simulink model "sys1"  (R2023b)
settings: Solver=VariableStepAuto  StartTime=0.0  StopTime=30e-3  RelTol=1e-3
InitFcn:
  | fs = 100e6;
  | ts = 1 / fs;
values from neighbouring files (symbols this model uses):
  c = 3e8    (= 300000000)    [init_param.m]
  H_az1 = zeros(numSamples,numPulses)    [init_param.m]
  H_az2 = zeros(numSamples,numPulses)    [init_param.m]
  H_ref = fft(conj(fliplr(txChirp)), numSamples)    [init_param.m]
  rawData = rawData + 0.01 * (randn(size(rawData)) + 1j * randn(size(rawData)))    [init_param.m]
  x1 = zeros(size(rawData))    [main.m]
  x2 = zeros(size(x1))    [main.m]
  x3 = zeros(size(x2))    [main.m]
  x4 = zeros(size(x3))    [main.m]
  x5 = zeros(size(x4))    [main.m]
  x6 = zeros(size(x5))    [main.m]
  xx4 = zeros(size(xx3))    [main.m]
  xx5 = zeros(size(xx4))    [main.m]
  xx6 = zeros(size(xx5))    [main.m]
undefined symbols (not defined in the file or in its folder): ffva1156, w2, w3, w4, w5, w6, w7, w8, w9, ww2, ww3, ww4, ww5, ww6, ww7, ww8, ww9, xcku095
libraries: hdlBasic x917, hdlDSPIP x18, dspsrcs4 x12, vmcUtilities x1
(part 2 of 9)

== system sys1/SAR/stream/stream_ifft ==
  en : Inport
  re : Inport  Port=2
  im : Inport  Port=3
  Scale : hdlBasic/Scale  scale_factor=15  XmcBlockStatus=1  maskContainerNames=group1  block_type=scale  block_config=sysgen:Scale_config
  Scale1 : hdlBasic/Scale  scale_factor=15  XmcBlockStatus=1  maskContainerNames=group1  block_type=scale  block_config=sysgen:Scale_config
  Scale2 : hdlBasic/Scale  scale_factor=-15  XmcBlockStatus=1  maskContainerNames=group1  block_type=scale  block_config=sysgen:Scale_config
  Scale3 : hdlBasic/Scale  scale_factor=-15  XmcBlockStatus=1  maskContainerNames=group1  block_type=scale  block_config=sysgen:Scale_config
  stage1 : Subsystem
  stage2 : Subsystem
  stage3 : Subsystem
  stage4 : Subsystem
  stage5 : Subsystem
  stage6 : Subsystem
  stage7 : Subsystem
  stage8 : Subsystem
  stage9 : Subsystem
  valid : Outport
  out_re : Outport  Port=2
  out_im : Outport  Port=3
  wires:
  stage7/3(out_im) -> stage8/3(im)
  stage5/3(out_im) -> stage6/3(im)
  stage8/3(out_im) -> stage9/3(im)
  en/1 -> stage1/1(en)
  stage2/3(out_im) -> stage3/3(im)
  stage1/3(out_im) -> stage2/3(im)
  stage6/3(out_im) -> stage7/3(im)
  stage4/3(out_im) -> stage5/3(im)
  im/1 -> Scale1/1
  stage3/3(out_im) -> stage4/3(im)
  re/1 -> Scale/1
  stage9/3(out_im) -> Scale3/1
  stage1/1(valid) -> stage2/1(en)
  stage1/2(out_re) -> stage2/2(re)
  stage2/2(out_re) -> stage3/2(re)
  stage2/1(valid) -> stage3/1(en)
  stage3/1(valid) -> stage4/1(en)
  stage3/2(out_re) -> stage4/2(re)
  stage4/2(out_re) -> stage5/2(re)
  stage4/1(valid) -> stage5/1(en)
  stage5/1(valid) -> stage6/1(en)
  stage5/2(out_re) -> stage6/2(re)
  stage6/2(out_re) -> stage7/2(re)
  stage6/1(valid) -> stage7/1(en)
  stage7/1(valid) -> stage8/1(en)
  stage7/2(out_re) -> stage8/2(re)
  stage8/2(out_re) -> stage9/2(re)
  stage8/1(valid) -> stage9/1(en)
  stage9/1(valid) -> valid/1
  stage9/2(out_re) -> Scale2/1
  Scale/1 -> stage1/2(re)
  Scale1/1 -> stage1/3(im)
  Scale2/1 -> out_re/1
  Scale3/1 -> out_im/1

== system sys1/SAR/stream/stream_fft/stage1 ==
  en : Inport
  re : Inport  Port=2
  im : Inport  Port=3
  BF : Subsystem
      settings: PortSchema="{\"entries\":[{\"content\":{\"sides\":[{\"content\":{\"connectorIds\":[\"In1\",\"In2\",\"Out3\",\"Out4\"]},\"type\":\"ConnectorPlacement.EquallySpacedRectSide\",\"uuid\":\"dc9f2664-179f-4a56-867a-12fe61ba91e8\"},{\"content\":{\"connectorIds\":[\"Out1\",\"Out2\",\"In3\",\"In4\"],\"side\":\"RIGHT\"},\"type\":\"ConnectorPlacement.EquallySpacedRectSide\",\"uuid\":\"0b440064-4d1a-4bb1-bd44-91090294f336\"},{\"content\":{\"side\":\"TOP\"},\"type\":\"ConnectorPlacement.EquallySpacedRectSide\",\"uuid\":\"bf93b41b-a3ae-4711-be50-aae2b8452a00\"}]},\"type\":\"ConnectorPlacement.EquallySpacedConnector\",\"uuid\":\"12001bad-0a53-45ef-b6ab-2c1b34cc57fa\"}],\"packageUris\":[\"http://schema.mathworks.com/mf0/Connector/R2020b\"],\"version\":\"1.0\"}"
  Constant : hdlBasic/Constant  const=2^10  gui_display_data_type=Fixed-point  arith_type=Unsigned  n_bits=20  bin_pt=0  preci_type=Single  exp_width=8  frac_width=24  explicit_period=off  period=1  XmcBlockStatus=1  maskContainerNames=tabcontainer1  block_type=constant  block_config=sysgen:Constant_config
  Constant1 : hdlBasic/Constant  const=1  gui_display_data_type=Boolean  arith_type=Boolean  n_bits=16  bin_pt=14  preci_type=Single  exp_width=8  frac_width=24  explicit_period=on  period=ts  XmcBlockStatus=1  maskContainerNames=tabcontainer1  block_type=constant  block_config=sysgen:Constant_config
  Counter1 : hdlBasic/Counter  cnt_type=Free running  cnt_to=Inf  operation=Up  start_count=0  cnt_by_val=1  arith_type=Unsigned  n_bits=20  bin_pt=0  load_pin=off  rst=off  en=on  explicit_period=Explicit  period=ts  use_behavioral_HDL=off  implementation=Fabric  XmcBlockStatus=1  maskContainerNames=group1  block_type=counter  block_config=sysgen:Counter_config  block_width=531  block_height=1023
  Delay1 : hdlBasic/Delay  rst=off  en=off  latency=6  reg_retiming=off  XmcBlockStatus=1  maskContainerNames=group1  block_type=delay  block_config=sysgen:Delay_config
  Delay4 : hdlBasic/Delay  rst=off  en=off  latency=7  reg_retiming=off  XmcBlockStatus=1  maskContainerNames=group1  block_type=delay  block_config=sysgen:Delay_config
  Multiplexer : Subsystem
      settings: PortSchema="{\"entries\":[{\"content\":{\"sides\":[{\"content\":{\"connectorIds\":[\"In1\",\"In2\",\"In3\",\"In4\"]},\"type\":\"ConnectorPlacement.EquallySpacedRectSide\",\"uuid\":\"d39b2674-e61f-4632-a918-ea673b128ff5\"},{\"content\":{\"connectorIds\":[\"Out1\",\"Out2\"],\"side\":\"RIGHT\"},\"type\":\"ConnectorPlacement.EquallySpacedRectSide\",\"uuid\":\"03c9bc0a-e0d2-45eb-9b7a-9d06bc1b3e13\"},{\"content\":{\"connectorIds\":[\"In5\"],\"side\":\"TOP\"},\"type\":\"ConnectorPlacement.EquallySpacedRectSide\",\"uuid\":\"49e788e0-ebb0-431e-96ea-edf312796710\"}]},\"type\":\"ConnectorPlacement.EquallySpacedConnector\",\"uuid\":\"eef61444-07bb-4ce5-a4f8-b8563d493c59\"}],\"packageUris\":[\"http://schema.mathworks.com/mf0/Connector/R2020b\"],\"version\":\"1.0\"}"
  Register2 : hdlBasic/Register  init=0  rst=off  en=on  XmcBlockStatus=1  maskContainerNames=tabcontainer1  block_type=register  block_config=sysgen:Register_config
  Relational : hdlBasic/Relational  mode=a=b  op_type=Bool  en=off  latency=0  XmcBlockStatus=1  maskContainerNames=tabcontainer1  block_type=relational  block_config=sysgen:Relational_config
  Shift2 : hdlBasic/Shift  shift_dir=Right  shift_bits=1  en=off  latency=0  precision=User Defined  arith_type="Signed  (2's comp)"  n_bits=16  bin_pt=0  quantization="Round  (unbiased: +/- Inf)"  overflow=Flag as error  XmcBlockStatus=1  maskContainerNames=group2  block_type=shift  block_config=sysgen:Shift_config
  Shift3 : hdlBasic/Shift  shift_dir=Right  shift_bits=1  en=off  latency=0  precision=User Defined  arith_type="Signed  (2's comp)"  n_bits=16  bin_pt=0  quantization="Round  (unbiased: +/- Inf)"  overflow=Flag as error  XmcBlockStatus=1  maskContainerNames=group2  block_type=shift  block_config=sysgen:Shift_config
  Twiddle : Subsystem
      settings: PortSchema="{\"entries\":[{\"content\":{\"sides\":[{\"content\":{\"connectorIds\":[\"In1\",\"In2\"]},\"type\":\"ConnectorPlacement.EquallySpacedRectSide\",\"uuid\":\"ecfcc33a-c00e-4245-880a-d3e35376b375\"},{\"content\":{\"connectorIds\":[\"Out1\",\"Out2\"],\"side\":\"RIGHT\"},\"type\":\"ConnectorPlacement.EquallySpacedRectSide\",\"uuid\":\"26b6cb3a-d864-4641-9d64-3816f5e3e677\"},{\"content\":{\"connectorIds\":[\"In3\"],\"side\":\"TOP\"},\"type\":\"ConnectorPlacement.EquallySpacedRectSide\",\"uuid\":\"0115c513-98ce-476e-a096-a4849d96f6f0\"}]},\"type\":\"ConnectorPlacement.EquallySpacedConnector\",\"uuid\":\"ace197b1-74a9-4d2b-80b6-f8336c43cac2\"}],\"packageUris\":[\"http://schema.mathworks.com/mf0/Connector/R2020b\"],\"version\":\"1.0\"}"
  delay : Subsystem
      settings: PortSchema="{\"entries\":[{\"content\":{\"sides\":[{\"content\":{\"connectorIds\":[\"In1\",\"In2\"]},\"type\":\"ConnectorPlacement.EquallySpacedRectSide\",\"uuid\":\"ba2590db-591f-426e-a159-0b5b6e6f2a83\"},{\"content\":{\"connectorIds\":[\"Out1\",\"Out2\",\"In4\",\"In5\"],\"side\":\"RIGHT\"},\"type\":\"ConnectorPlacement.EquallySpacedRectSide\",\"uuid\":\"3a7188c9-1b60-4adb-8ab5-3e5ce503b358\"},{\"content\":{\"connectorIds\":[\"In3\"],\"side\":\"TOP\"},\"type\":\"ConnectorPlacement.EquallySpacedRectSide\",\"uuid\":\"d7972a41-1a3e-4417-8334-615e53660bc0\"}]},\"type\":\"ConnectorPlacement.EquallySpacedConnector\",\"uuid\":\"9fe28d71-4153-49dc-89fd-80824351344f\"}],\"packageUris\":[\"http://schema.mathworks.com/mf0/Connector/R2020b\"],\"version\":\"1.0\"}"
  valid : Outport
  out_re : Outport  Port=2
  out_im : Outport  Port=3
  wires:
  Shift3/1 -> delay/2(i), BF/4(im1)
  Shift2/1 -> delay/1(r), BF/3(re1)
  en/1 -> Counter1/1
  Constant/1 -> Relational/2
  Relational/1 -> Register2/2
  Constant1/1 -> Register2/1
  delay/1(rr) -> BF/1(re2), Twiddle/1(r)
  delay/2(ii) -> BF/2(im2), Twiddle/2(i)
  BF/3(Out1_r) -> delay/4(r1)
  BF/4(Out1_i) -> delay/5(i1)
  Register2/1 -> Delay1/1
  Counter1/1 -> Relational/1, Delay4/1, Twiddle/3(cnt), delay/3(cnt)
  re/1 -> Shift2/1
  im/1 -> Shift3/1
  Twiddle/1(rr) -> Multiplexer/1(r1)
  Twiddle/2(ii) -> Multiplexer/2(i1)
  BF/1(Out2_r) -> Multiplexer/3(r2)
  BF/2(Out2_i) -> Multiplexer/4(i2)
  Delay4/1 -> Multiplexer/5(cnt)
  Multiplexer/1(rr) -> out_re/1
  Multiplexer/2(ii) -> out_im/1
  Delay1/1 -> valid/1

== system sys1/SAR/stream/stream_fft/stage2 ==
  en : Inport
  re : Inport  Port=2
  im : Inport  Port=3
  BF : Subsystem
      settings: PortSchema="{\"entries\":[{\"content\":{\"sides\":[{\"content\":{\"connectorIds\":[\"In1\",\"In2\",\"Out3\",\"Out4\"]},\"type\":\"ConnectorPlacement.EquallySpacedRectSide\",\"uuid\":\"dc9f2664-179f-4a56-867a-12fe61ba91e8\"},{\"content\":{\"connectorIds\":[\"Out1\",\"Out2\",\"In3\",\"In4\"],\"side\":\"RIGHT\"},\"type\":\"ConnectorPlacement.EquallySpacedRectSide\",\"uuid\":\"0b440064-4d1a-4bb1-bd44-91090294f336\"},{\"content\":{\"side\":\"TOP\"},\"type\":\"ConnectorPlacement.EquallySpacedRectSide\",\"uuid\":\"bf93b41b-a3ae-4711-be50-aae2b8452a00\"}]},\"type\":\"ConnectorPlacement.EquallySpacedConnector\",\"uuid\":\"12001bad-0a53-45ef-b6ab-2c1b34cc57fa\"}],\"packageUris\":[\"http://schema.mathworks.com/mf0/Connector/R2020b\"],\"version\":\"1.0\"}"
  Constant : hdlBasic/Constant  const=2^11  gui_display_data_type=Fixed-point  arith_type=Unsigned  n_bits=20  bin_pt=0  preci_type=Single  exp_width=8  frac_width=24  explicit_period=off  period=1  XmcBlockStatus=1  maskContainerNames=tabcontainer1  block_type=constant  block_config=sysgen:Constant_config
  Constant1 : hdlBasic/Constant  const=1  gui_display_data_type=Boolean  arith_type=Boolean  n_bits=16  bin_pt=14  preci_type=Single  exp_width=8  frac_width=24  explicit_period=on  period=ts  XmcBlockStatus=1  maskContainerNames=tabcontainer1  block_type=constant  block_config=sysgen:Constant_config
  Counter1 : hdlBasic/Counter  cnt_type=Free running  cnt_to=Inf  operation=Up  start_count=0  cnt_by_val=1  arith_type=Unsigned  n_bits=20  bin_pt=0  load_pin=off  rst=off  en=on  explicit_period=Explicit  period=ts  use_behavioral_HDL=off  implementation=Fabric  XmcBlockStatus=1  maskContainerNames=group1  block_type=counter  block_config=sysgen:Counter_config  block_width=531  block_height=1023
  Delay1 : hdlBasic/Delay  rst=off  en=off  latency=6  reg_retiming=off  XmcBlockStatus=1  maskContainerNames=group1  block_type=delay  block_config=sysgen:Delay_config
  Delay4 : hdlBasic/Delay  rst=off  en=off  latency=7  reg_retiming=off  XmcBlockStatus=1  maskContainerNames=group1  block_type=delay  block_config=sysgen:Delay_config
  Multiplexer : Subsystem
      settings: PortSchema="{\"entries\":[{\"content\":{\"sides\":[{\"content\":{\"connectorIds\":[\"In1\",\"In2\",\"In3\",\"In4\"]},\"type\":\"ConnectorPlacement.EquallySpacedRectSide\",\"uuid\":\"d39b2674-e61f-4632-a918-ea673b128ff5\"},{\"content\":{\"connectorIds\":[\"Out1\",\"Out2\"],\"side\":\"RIGHT\"},\"type\":\"ConnectorPlacement.EquallySpacedRectSide\",\"uuid\":\"03c9bc0a-e0d2-45eb-9b7a-9d06bc1b3e13\"},{\"content\":{\"connectorIds\":[\"In5\"],\"side\":\"TOP\"},\"type\":\"ConnectorPlacement.EquallySpacedRectSide\",\"uuid\":\"49e788e0-ebb0-431e-96ea-edf312796710\"}]},\"type\":\"ConnectorPlacement.EquallySpacedConnector\",\"uuid\":\"eef61444-07bb-4ce5-a4f8-b8563d493c59\"}],\"packageUris\":[\"http://schema.mathworks.com/mf0/Connector/R2020b\"],\"version\":\"1.0\"}"
  Register2 : hdlBasic/Register  init=0  rst=off  en=on  XmcBlockStatus=1  maskContainerNames=tabcontainer1  block_type=register  block_config=sysgen:Register_config
  Relational : hdlBasic/Relational  mode=a=b  op_type=Bool  en=off  latency=0  XmcBlockStatus=1  maskContainerNames=tabcontainer1  block_type=relational  block_config=sysgen:Relational_config
  Shift2 : hdlBasic/Shift  shift_dir=Right  shift_bits=1  en=off  latency=0  precision=User Defined  arith_type="Signed  (2's comp)"  n_bits=16  bin_pt=0  quantization="Round  (unbiased: +/- Inf)"  overflow=Flag as error  XmcBlockStatus=1  maskContainerNames=group2  block_type=shift  block_config=sysgen:Shift_config
  Shift3 : hdlBasic/Shift  shift_dir=Right  shift_bits=1  en=off  latency=0  precision=User Defined  arith_type="Signed  (2's comp)"  n_bits=16  bin_pt=0  quantization="Round  (unbiased: +/- Inf)"  overflow=Flag as error  XmcBlockStatus=1  maskContainerNames=group2  block_type=shift  block_config=sysgen:Shift_config
  Twiddle : Subsystem
      settings: PortSchema="{\"entries\":[{\"content\":{\"sides\":[{\"content\":{\"connectorIds\":[\"In1\",\"In2\"]},\"type\":\"ConnectorPlacement.EquallySpacedRectSide\",\"uuid\":\"ecfcc33a-c00e-4245-880a-d3e35376b375\"},{\"content\":{\"connectorIds\":[\"Out1\",\"Out2\"],\"side\":\"RIGHT\"},\"type\":\"ConnectorPlacement.EquallySpacedRectSide\",\"uuid\":\"26b6cb3a-d864-4641-9d64-3816f5e3e677\"},{\"content\":{\"connectorIds\":[\"In3\"],\"side\":\"TOP\"},\"type\":\"ConnectorPlacement.EquallySpacedRectSide\",\"uuid\":\"0115c513-98ce-476e-a096-a4849d96f6f0\"}]},\"type\":\"ConnectorPlacement.EquallySpacedConnector\",\"uuid\":\"ace197b1-74a9-4d2b-80b6-f8336c43cac2\"}],\"packageUris\":[\"http://schema.mathworks.com/mf0/Connector/R2020b\"],\"version\":\"1.0\"}"
  delay : Subsystem
      settings: PortSchema="{\"entries\":[{\"content\":{\"sides\":[{\"content\":{\"connectorIds\":[\"In1\",\"In2\"]},\"type\":\"ConnectorPlacement.EquallySpacedRectSide\",\"uuid\":\"ba2590db-591f-426e-a159-0b5b6e6f2a83\"},{\"content\":{\"connectorIds\":[\"Out1\",\"Out2\",\"In4\",\"In5\"],\"side\":\"RIGHT\"},\"type\":\"ConnectorPlacement.EquallySpacedRectSide\",\"uuid\":\"3a7188c9-1b60-4adb-8ab5-3e5ce503b358\"},{\"content\":{\"connectorIds\":[\"In3\"],\"side\":\"TOP\"},\"type\":\"ConnectorPlacement.EquallySpacedRectSide\",\"uuid\":\"d7972a41-1a3e-4417-8334-615e53660bc0\"}]},\"type\":\"ConnectorPlacement.EquallySpacedConnector\",\"uuid\":\"9fe28d71-4153-49dc-89fd-80824351344f\"}],\"packageUris\":[\"http://schema.mathworks.com/mf0/Connector/R2020b\"],\"version\":\"1.0\"}"
  valid : Outport
  out_re : Outport  Port=2
  out_im : Outport  Port=3
  wires:
  Shift3/1 -> BF/4(im1), delay/2(i)
  Shift2/1 -> BF/3(re1), delay/1(r)
  Delay1/1 -> valid/1
  Multiplexer/2(ii) -> out_im/1
  Multiplexer/1(rr) -> out_re/1
  Delay4/1 -> Multiplexer/5(cnt)
  BF/2(Out2_i) -> Multiplexer/4(i2)
  BF/1(Out2_r) -> Multiplexer/3(r2)
  Twiddle/2(ii) -> Multiplexer/2(i1)
  Twiddle/1(rr) -> Multiplexer/1(r1)
  im/1 -> Shift3/1
  re/1 -> Shift2/1
  Counter1/1 -> delay/3(cnt), Twiddle/3(cnt), Delay4/1, Relational/1
  Register2/1 -> Delay1/1
  BF/4(Out1_i) -> delay/5(i1)
  BF/3(Out1_r) -> delay/4(r1)
  delay/2(ii) -> Twiddle/2(i), BF/2(im2)
  delay/1(rr) -> Twiddle/1(r), BF/1(re2)
  Constant1/1 -> Register2/1
  Relational/1 -> Register2/2
  Constant/1 -> Relational/2
  en/1 -> Counter1/1

== system sys1/SAR/stream/stream_fft/stage3 ==
  en : Inport
  re : Inport  Port=2
  im : Inport  Port=3
  BF : Subsystem
      settings: PortSchema="{\"entries\":[{\"content\":{\"sides\":[{\"content\":{\"connectorIds\":[\"In1\",\"In2\",\"Out3\",\"Out4\"]},\"type\":\"ConnectorPlacement.EquallySpacedRectSide\",\"uuid\":\"dc9f2664-179f-4a56-867a-12fe61ba91e8\"},{\"content\":{\"connectorIds\":[\"Out1\",\"Out2\",\"In3\",\"In4\"],\"side\":\"RIGHT\"},\"type\":\"ConnectorPlacement.EquallySpacedRectSide\",\"uuid\":\"0b440064-4d1a-4bb1-bd44-91090294f336\"},{\"content\":{\"side\":\"TOP\"},\"type\":\"ConnectorPlacement.EquallySpacedRectSide\",\"uuid\":\"bf93b41b-a3ae-4711-be50-aae2b8452a00\"}]},\"type\":\"ConnectorPlacement.EquallySpacedConnector\",\"uuid\":\"12001bad-0a53-45ef-b6ab-2c1b34cc57fa\"}],\"packageUris\":[\"http://schema.mathworks.com/mf0/Connector/R2020b\"],\"version\":\"1.0\"}"
  Constant : hdlBasic/Constant  const=2^12  gui_display_data_type=Fixed-point  arith_type=Unsigned  n_bits=20  bin_pt=0  preci_type=Single  exp_width=8  frac_width=24  explicit_period=off  period=1  XmcBlockStatus=1  maskContainerNames=tabcontainer1  block_type=constant  block_config=sysgen:Constant_config
  Constant1 : hdlBasic/Constant  const=1  gui_display_data_type=Boolean  arith_type=Boolean  n_bits=16  bin_pt=14  preci_type=Single  exp_width=8  frac_width=24  explicit_period=on  period=ts  XmcBlockStatus=1  maskContainerNames=tabcontainer1  block_type=constant  block_config=sysgen:Constant_config
  Counter1 : hdlBasic/Counter  cnt_type=Free running  cnt_to=Inf  operation=Up  start_count=0  cnt_by_val=1  arith_type=Unsigned  n_bits=20  bin_pt=0  load_pin=off  rst=off  en=on  explicit_period=Explicit  period=ts  use_behavioral_HDL=off  implementation=Fabric  XmcBlockStatus=1  maskContainerNames=group1  block_type=counter  block_config=sysgen:Counter_config  block_width=531  block_height=1023
  Delay1 : hdlBasic/Delay  rst=off  en=off  latency=6  reg_retiming=off  XmcBlockStatus=1  maskContainerNames=group1  block_type=delay  block_config=sysgen:Delay_config
  Delay4 : hdlBasic/Delay  rst=off  en=off  latency=7  reg_retiming=off  XmcBlockStatus=1  maskContainerNames=group1  block_type=delay  block_config=sysgen:Delay_config
  Multiplexer : Subsystem
      settings: PortSchema="{\"entries\":[{\"content\":{\"sides\":[{\"content\":{\"connectorIds\":[\"In1\",\"In2\",\"In3\",\"In4\"]},\"type\":\"ConnectorPlacement.EquallySpacedRectSide\",\"uuid\":\"d39b2674-e61f-4632-a918-ea673b128ff5\"},{\"content\":{\"connectorIds\":[\"Out1\",\"Out2\"],\"side\":\"RIGHT\"},\"type\":\"ConnectorPlacement.EquallySpacedRectSide\",\"uuid\":\"03c9bc0a-e0d2-45eb-9b7a-9d06bc1b3e13\"},{\"content\":{\"connectorIds\":[\"In5\"],\"side\":\"TOP\"},\"type\":\"ConnectorPlacement.EquallySpacedRectSide\",\"uuid\":\"49e788e0-ebb0-431e-96ea-edf312796710\"}]},\"type\":\"ConnectorPlacement.EquallySpacedConnector\",\"uuid\":\"eef61444-07bb-4ce5-a4f8-b8563d493c59\"}],\"packageUris\":[\"http://schema.mathworks.com/mf0/Connector/R2020b\"],\"version\":\"1.0\"}"
  Register2 : hdlBasic/Register  init=0  rst=off  en=on  XmcBlockStatus=1  maskContainerNames=tabcontainer1  block_type=register  block_config=sysgen:Register_config
  Relational : hdlBasic/Relational  mode=a=b  op_type=Bool  en=off  latency=0  XmcBlockStatus=1  maskContainerNames=tabcontainer1  block_type=relational  block_config=sysgen:Relational_config
  Shift2 : hdlBasic/Shift  shift_dir=Right  shift_bits=1  en=off  latency=0  precision=User Defined  arith_type="Signed  (2's comp)"  n_bits=16  bin_pt=0  quantization="Round  (unbiased: +/- Inf)"  overflow=Flag as error  XmcBlockStatus=1  maskContainerNames=group2  block_type=shift  block_config=sysgen:Shift_config
  Shift3 : hdlBasic/Shift  shift_dir=Right  shift_bits=1  en=off  latency=0  precision=User Defined  arith_type="Signed  (2's comp)"  n_bits=16  bin_pt=0  quantization="Round  (unbiased: +/- Inf)"  overflow=Flag as error  XmcBlockStatus=1  maskContainerNames=group2  block_type=shift  block_config=sysgen:Shift_config
  Twiddle : Subsystem
      settings: PortSchema="{\"entries\":[{\"content\":{\"sides\":[{\"content\":{\"connectorIds\":[\"In1\",\"In2\"]},\"type\":\"ConnectorPlacement.EquallySpacedRectSide\",\"uuid\":\"ecfcc33a-c00e-4245-880a-d3e35376b375\"},{\"content\":{\"connectorIds\":[\"Out1\",\"Out2\"],\"side\":\"RIGHT\"},\"type\":\"ConnectorPlacement.EquallySpacedRectSide\",\"uuid\":\"26b6cb3a-d864-4641-9d64-3816f5e3e677\"},{\"content\":{\"connectorIds\":[\"In3\"],\"side\":\"TOP\"},\"type\":\"ConnectorPlacement.EquallySpacedRectSide\",\"uuid\":\"0115c513-98ce-476e-a096-a4849d96f6f0\"}]},\"type\":\"ConnectorPlacement.EquallySpacedConnector\",\"uuid\":\"ace197b1-74a9-4d2b-80b6-f8336c43cac2\"}],\"packageUris\":[\"http://schema.mathworks.com/mf0/Connector/R2020b\"],\"version\":\"1.0\"}"
  delay : Subsystem
      settings: PortSchema="{\"entries\":[{\"content\":{\"sides\":[{\"content\":{\"connectorIds\":[\"In1\",\"In2\"]},\"type\":\"ConnectorPlacement.EquallySpacedRectSide\",\"uuid\":\"ba2590db-591f-426e-a159-0b5b6e6f2a83\"},{\"content\":{\"connectorIds\":[\"Out1\",\"Out2\",\"In4\",\"In5\"],\"side\":\"RIGHT\"},\"type\":\"ConnectorPlacement.EquallySpacedRectSide\",\"uuid\":\"3a7188c9-1b60-4adb-8ab5-3e5ce503b358\"},{\"content\":{\"connectorIds\":[\"In3\"],\"side\":\"TOP\"},\"type\":\"ConnectorPlacement.EquallySpacedRectSide\",\"uuid\":\"d7972a41-1a3e-4417-8334-615e53660bc0\"}]},\"type\":\"ConnectorPlacement.EquallySpacedConnector\",\"uuid\":\"9fe28d71-4153-49dc-89fd-80824351344f\"}],\"packageUris\":[\"http://schema.mathworks.com/mf0/Connector/R2020b\"],\"version\":\"1.0\"}"
  valid : Outport
  out_re : Outport  Port=2
  out_im : Outport  Port=3
  wires:
  Shift3/1 -> delay/2(i), BF/4(im1)
  Shift2/1 -> delay/1(r), BF/3(re1)
  en/1 -> Counter1/1
  Constant/1 -> Relational/2
  Relational/1 -> Register2/2
  Constant1/1 -> Register2/1
  delay/1(rr) -> BF/1(re2), Twiddle/1(r)
  delay/2(ii) -> BF/2(im2), Twiddle/2(i)
  BF/3(Out1_r) -> delay/4(r1)
  BF/4(Out1_i) -> delay/5(i1)
  Register2/1 -> Delay1/1
  Counter1/1 -> Relational/1, Delay4/1, Twiddle/3(cnt), delay/3(cnt)
  re/1 -> Shift2/1
  im/1 -> Shift3/1
  Twiddle/1(rr) -> Multiplexer/1(r1)
  Twiddle/2(ii) -> Multiplexer/2(i1)
  BF/1(Out2_r) -> Multiplexer/3(r2)
  BF/2(Out2_i) -> Multiplexer/4(i2)
  Delay4/1 -> Multiplexer/5(cnt)
  Multiplexer/1(rr) -> out_re/1
  Multiplexer/2(ii) -> out_im/1
  Delay1/1 -> valid/1

== system sys1/SAR/stream/stream_fft/stage4 ==
  en : Inport
  re : Inport  Port=2
  im : Inport  Port=3
  BF : Subsystem
      settings: PortSchema="{\"entries\":[{\"content\":{\"sides\":[{\"content\":{\"connectorIds\":[\"In1\",\"In2\",\"Out3\",\"Out4\"]},\"type\":\"ConnectorPlacement.EquallySpacedRectSide\",\"uuid\":\"dc9f2664-179f-4a56-867a-12fe61ba91e8\"},{\"content\":{\"connectorIds\":[\"Out1\",\"Out2\",\"In3\",\"In4\"],\"side\":\"RIGHT\"},\"type\":\"ConnectorPlacement.EquallySpacedRectSide\",\"uuid\":\"0b440064-4d1a-4bb1-bd44-91090294f336\"},{\"content\":{\"side\":\"TOP\"},\"type\":\"ConnectorPlacement.EquallySpacedRectSide\",\"uuid\":\"bf93b41b-a3ae-4711-be50-aae2b8452a00\"}]},\"type\":\"ConnectorPlacement.EquallySpacedConnector\",\"uuid\":\"12001bad-0a53-45ef-b6ab-2c1b34cc57fa\"}],\"packageUris\":[\"http://schema.mathworks.com/mf0/Connector/R2020b\"],\"version\":\"1.0\"}"
  Constant : hdlBasic/Constant  const=2^13  gui_display_data_type=Fixed-point  arith_type=Unsigned  n_bits=20  bin_pt=0  preci_type=Single  exp_width=8  frac_width=24  explicit_period=off  period=1  XmcBlockStatus=1  maskContainerNames=tabcontainer1  block_type=constant  block_config=sysgen:Constant_config
  Constant1 : hdlBasic/Constant  const=1  gui_display_data_type=Boolean  arith_type=Boolean  n_bits=16  bin_pt=14  preci_type=Single  exp_width=8  frac_width=24  explicit_period=on  period=ts  XmcBlockStatus=1  maskContainerNames=tabcontainer1  block_type=constant  block_config=sysgen:Constant_config
  Counter1 : hdlBasic/Counter  cnt_type=Free running  cnt_to=Inf  operation=Up  start_count=0  cnt_by_val=1  arith_type=Unsigned  n_bits=20  bin_pt=0  load_pin=off  rst=off  en=on  explicit_period=Explicit  period=ts  use_behavioral_HDL=off  implementation=Fabric  XmcBlockStatus=1  maskContainerNames=group1  block_type=counter  block_config=sysgen:Counter_config  block_width=531  block_height=1023
  Delay1 : hdlBasic/Delay  rst=off  en=off  latency=6  reg_retiming=off  XmcBlockStatus=1  maskContainerNames=group1  block_type=delay  block_config=sysgen:Delay_config
  Delay4 : hdlBasic/Delay  rst=off  en=off  latency=7  reg_retiming=off  XmcBlockStatus=1  maskContainerNames=group1  block_type=delay  block_config=sysgen:Delay_config
  Multiplexer : Subsystem
      settings: PortSchema="{\"entries\":[{\"content\":{\"sides\":[{\"content\":{\"connectorIds\":[\"In1\",\"In2\",\"In3\",\"In4\"]},\"type\":\"ConnectorPlacement.EquallySpacedRectSide\",\"uuid\":\"d39b2674-e61f-4632-a918-ea673b128ff5\"},{\"content\":{\"connectorIds\":[\"Out1\",\"Out2\"],\"side\":\"RIGHT\"},\"type\":\"ConnectorPlacement.EquallySpacedRectSide\",\"uuid\":\"03c9bc0a-e0d2-45eb-9b7a-9d06bc1b3e13\"},{\"content\":{\"connectorIds\":[\"In5\"],\"side\":\"TOP\"},\"type\":\"ConnectorPlacement.EquallySpacedRectSide\",\"uuid\":\"49e788e0-ebb0-431e-96ea-edf312796710\"}]},\"type\":\"ConnectorPlacement.EquallySpacedConnector\",\"uuid\":\"eef61444-07bb-4ce5-a4f8-b8563d493c59\"}],\"packageUris\":[\"http://schema.mathworks.com/mf0/Connector/R2020b\"],\"version\":\"1.0\"}"
  Register2 : hdlBasic/Register  init=0  rst=off  en=on  XmcBlockStatus=1  maskContainerNames=tabcontainer1  block_type=register  block_config=sysgen:Register_config
  Relational : hdlBasic/Relational  mode=a=b  op_type=Bool  en=off  latency=0  XmcBlockStatus=1  maskContainerNames=tabcontainer1  block_type=relational  block_config=sysgen:Relational_config
  Shift2 : hdlBasic/Shift  shift_dir=Right  shift_bits=1  en=off  latency=0  precision=User Defined  arith_type="Signed  (2's comp)"  n_bits=16  bin_pt=0  quantization="Round  (unbiased: +/- Inf)"  overflow=Flag as error  XmcBlockStatus=1  maskContainerNames=group2  block_type=shift  block_config=sysgen:Shift_config
  Shift3 : hdlBasic/Shift  shift_dir=Right  shift_bits=1  en=off  latency=0  precision=User Defined  arith_type="Signed  (2's comp)"  n_bits=16  bin_pt=0  quantization="Round  (unbiased: +/- Inf)"  overflow=Flag as error  XmcBlockStatus=1  maskContainerNames=group2  block_type=shift  block_config=sysgen:Shift_config
  Twiddle : Subsystem
      settings: PortSchema="{\"entries\":[{\"content\":{\"sides\":[{\"content\":{\"connectorIds\":[\"In1\",\"In2\"]},\"type\":\"ConnectorPlacement.EquallySpacedRectSide\",\"uuid\":\"ecfcc33a-c00e-4245-880a-d3e35376b375\"},{\"content\":{\"connectorIds\":[\"Out1\",\"Out2\"],\"side\":\"RIGHT\"},\"type\":\"ConnectorPlacement.EquallySpacedRectSide\",\"uuid\":\"26b6cb3a-d864-4641-9d64-3816f5e3e677\"},{\"content\":{\"connectorIds\":[\"In3\"],\"side\":\"TOP\"},\"type\":\"ConnectorPlacement.EquallySpacedRectSide\",\"uuid\":\"0115c513-98ce-476e-a096-a4849d96f6f0\"}]},\"type\":\"ConnectorPlacement.EquallySpacedConnector\",\"uuid\":\"ace197b1-74a9-4d2b-80b6-f8336c43cac2\"}],\"packageUris\":[\"http://schema.mathworks.com/mf0/Connector/R2020b\"],\"version\":\"1.0\"}"
  delay : Subsystem
      settings: PortSchema="{\"entries\":[{\"content\":{\"sides\":[{\"content\":{\"connectorIds\":[\"In1\",\"In2\"]},\"type\":\"ConnectorPlacement.EquallySpacedRectSide\",\"uuid\":\"ba2590db-591f-426e-a159-0b5b6e6f2a83\"},{\"content\":{\"connectorIds\":[\"Out1\",\"Out2\",\"In4\",\"In5\"],\"side\":\"RIGHT\"},\"type\":\"ConnectorPlacement.EquallySpacedRectSide\",\"uuid\":\"3a7188c9-1b60-4adb-8ab5-3e5ce503b358\"},{\"content\":{\"connectorIds\":[\"In3\"],\"side\":\"TOP\"},\"type\":\"ConnectorPlacement.EquallySpacedRectSide\",\"uuid\":\"d7972a41-1a3e-4417-8334-615e53660bc0\"}]},\"type\":\"ConnectorPlacement.EquallySpacedConnector\",\"uuid\":\"9fe28d71-4153-49dc-89fd-80824351344f\"}],\"packageUris\":[\"http://schema.mathworks.com/mf0/Connector/R2020b\"],\"version\":\"1.0\"}"
  valid : Outport
  out_re : Outport  Port=2
  out_im : Outport  Port=3
  wires:
  Shift3/1 -> BF/4(im1), delay/2(i)
  Shift2/1 -> BF/3(re1), delay/1(r)
  Delay1/1 -> valid/1
  Multiplexer/2(ii) -> out_im/1
  Multiplexer/1(rr) -> out_re/1
  Delay4/1 -> Multiplexer/5(cnt)
  BF/2(Out2_i) -> Multiplexer/4(i2)
  BF/1(Out2_r) -> Multiplexer/3(r2)
  Twiddle/2(ii) -> Multiplexer/2(i1)
  Twiddle/1(rr) -> Multiplexer/1(r1)
  im/1 -> Shift3/1
  re/1 -> Shift2/1
  Counter1/1 -> delay/3(cnt), Twiddle/3(cnt), Delay4/1, Relational/1
  Register2/1 -> Delay1/1
  BF/4(Out1_i) -> delay/5(i1)
  BF/3(Out1_r) -> delay/4(r1)
  delay/2(ii) -> Twiddle/2(i), BF/2(im2)
  delay/1(rr) -> Twiddle/1(r), BF/1(re2)
  Constant1/1 -> Register2/1
  Relational/1 -> Register2/2
  Constant/1 -> Relational/2
  en/1 -> Counter1/1

== system sys1/SAR/stream/stream_fft/stage5 ==
  en : Inport
  re : Inport  Port=2
  im : Inport  Port=3
  BF : Subsystem
      settings: PortSchema="{\"entries\":[{\"content\":{\"sides\":[{\"content\":{\"connectorIds\":[\"In1\",\"In2\",\"Out3\",\"Out4\"]},\"type\":\"ConnectorPlacement.EquallySpacedRectSide\",\"uuid\":\"dc9f2664-179f-4a56-867a-12fe61ba91e8\"},{\"content\":{\"connectorIds\":[\"Out1\",\"Out2\",\"In3\",\"In4\"],\"side\":\"RIGHT\"},\"type\":\"ConnectorPlacement.EquallySpacedRectSide\",\"uuid\":\"0b440064-4d1a-4bb1-bd44-91090294f336\"},{\"content\":{\"side\":\"TOP\"},\"type\":\"ConnectorPlacement.EquallySpacedRectSide\",\"uuid\":\"bf93b41b-a3ae-4711-be50-aae2b8452a00\"}]},\"type\":\"ConnectorPlacement.EquallySpacedConnector\",\"uuid\":\"12001bad-0a53-45ef-b6ab-2c1b34cc57fa\"}],\"packageUris\":[\"http://schema.mathworks.com/mf0/Connector/R2020b\"],\"version\":\"1.0\"}"
  Constant : hdlBasic/Constant  const=2^14  gui_display_data_type=Fixed-point  arith_type=Unsigned  n_bits=20  bin_pt=0  preci_type=Single  exp_width=8  frac_width=24  explicit_period=off  period=1  XmcBlockStatus=1  maskContainerNames=tabcontainer1  block_type=constant  block_config=sysgen:Constant_config
  Constant1 : hdlBasic/Constant  const=1  gui_display_data_type=Boolean  arith_type=Boolean  n_bits=16  bin_pt=14  preci_type=Single  exp_width=8  frac_width=24  explicit_period=on  period=ts  XmcBlockStatus=1  maskContainerNames=tabcontainer1  block_type=constant  block_config=sysgen:Constant_config
  Counter1 : hdlBasic/Counter  cnt_type=Free running  cnt_to=Inf  operation=Up  start_count=0  cnt_by_val=1  arith_type=Unsigned  n_bits=20  bin_pt=0  load_pin=off  rst=off  en=on  explicit_period=Explicit  period=ts  use_behavioral_HDL=off  implementation=Fabric  XmcBlockStatus=1  maskContainerNames=group1  block_type=counter  block_config=sysgen:Counter_config  block_width=531  block_height=1023
  Delay1 : hdlBasic/Delay  rst=off  en=off  latency=6  reg_retiming=off  XmcBlockStatus=1  maskContainerNames=group1  block_type=delay  block_config=sysgen:Delay_config
  Delay4 : hdlBasic/Delay  rst=off  en=off  latency=7  reg_retiming=off  XmcBlockStatus=1  maskContainerNames=group1  block_type=delay  block_config=sysgen:Delay_config
  Multiplexer : Subsystem
      settings: PortSchema="{\"entries\":[{\"content\":{\"sides\":[{\"content\":{\"connectorIds\":[\"In1\",\"In2\",\"In3\",\"In4\"]},\"type\":\"ConnectorPlacement.EquallySpacedRectSide\",\"uuid\":\"d39b2674-e61f-4632-a918-ea673b128ff5\"},{\"content\":{\"connectorIds\":[\"Out1\",\"Out2\"],\"side\":\"RIGHT\"},\"type\":\"ConnectorPlacement.EquallySpacedRectSide\",\"uuid\":\"03c9bc0a-e0d2-45eb-9b7a-9d06bc1b3e13\"},{\"content\":{\"connectorIds\":[\"In5\"],\"side\":\"TOP\"},\"type\":\"ConnectorPlacement.EquallySpacedRectSide\",\"uuid\":\"49e788e0-ebb0-431e-96ea-edf312796710\"}]},\"type\":\"ConnectorPlacement.EquallySpacedConnector\",\"uuid\":\"eef61444-07bb-4ce5-a4f8-b8563d493c59\"}],\"packageUris\":[\"http://schema.mathworks.com/mf0/Connector/R2020b\"],\"version\":\"1.0\"}"
  Register2 : hdlBasic/Register  init=0  rst=off  en=on  XmcBlockStatus=1  maskContainerNames=tabcontainer1  block_type=register  block_config=sysgen:Register_config
  Relational : hdlBasic/Relational  mode=a=b  op_type=Bool  en=off  latency=0  XmcBlockStatus=1  maskContainerNames=tabcontainer1  block_type=relational  block_config=sysgen:Relational_config
  Shift2 : hdlBasic/Shift  shift_dir=Right  shift_bits=1  en=off  latency=0  precision=User Defined  arith_type="Signed  (2's comp)"  n_bits=16  bin_pt=0  quantization="Round  (unbiased: +/- Inf)"  overflow=Flag as error  XmcBlockStatus=1  maskContainerNames=group2  block_type=shift  block_config=sysgen:Shift_config
  Shift3 : hdlBasic/Shift  shift_dir=Right  shift_bits=1  en=off  latency=0  precision=User Defined  arith_type="Signed  (2's comp)"  n_bits=16  bin_pt=0  quantization="Round  (unbiased: +/- Inf)"  overflow=Flag as error  XmcBlockStatus=1  maskContainerNames=group2  block_type=shift  block_config=sysgen:Shift_config
  Twiddle : Subsystem
      settings: PortSchema="{\"entries\":[{\"content\":{\"sides\":[{\"content\":{\"connectorIds\":[\"In1\",\"In2\"]},\"type\":\"ConnectorPlacement.EquallySpacedRectSide\",\"uuid\":\"ecfcc33a-c00e-4245-880a-d3e35376b375\"},{\"content\":{\"connectorIds\":[\"Out1\",\"Out2\"],\"side\":\"RIGHT\"},\"type\":\"ConnectorPlacement.EquallySpacedRectSide\",\"uuid\":\"26b6cb3a-d864-4641-9d64-3816f5e3e677\"},{\"content\":{\"connectorIds\":[\"In3\"],\"side\":\"TOP\"},\"type\":\"ConnectorPlacement.EquallySpacedRectSide\",\"uuid\":\"0115c513-98ce-476e-a096-a4849d96f6f0\"}]},\"type\":\"ConnectorPlacement.EquallySpacedConnector\",\"uuid\":\"ace197b1-74a9-4d2b-80b6-f8336c43cac2\"}],\"packageUris\":[\"http://schema.mathworks.com/mf0/Connector/R2020b\"],\"version\":\"1.0\"}"
  delay : Subsystem
      settings: PortSchema="{\"entries\":[{\"content\":{\"sides\":[{\"content\":{\"connectorIds\":[\"In1\",\"In2\"]},\"type\":\"ConnectorPlacement.EquallySpacedRectSide\",\"uuid\":\"ba2590db-591f-426e-a159-0b5b6e6f2a83\"},{\"content\":{\"connectorIds\":[\"Out1\",\"Out2\",\"In4\",\"In5\"],\"side\":\"RIGHT\"},\"type\":\"ConnectorPlacement.EquallySpacedRectSide\",\"uuid\":\"3a7188c9-1b60-4adb-8ab5-3e5ce503b358\"},{\"content\":{\"connectorIds\":[\"In3\"],\"side\":\"TOP\"},\"type\":\"ConnectorPlacement.EquallySpacedRectSide\",\"uuid\":\"d7972a41-1a3e-4417-8334-615e53660bc0\"}]},\"type\":\"ConnectorPlacement.EquallySpacedConnector\",\"uuid\":\"9fe28d71-4153-49dc-89fd-80824351344f\"}],\"packageUris\":[\"http://schema.mathworks.com/mf0/Connector/R2020b\"],\"version\":\"1.0\"}"
  valid : Outport
  out_re : Outport  Port=2
  out_im : Outport  Port=3
  wires:
  Shift3/1 -> delay/2(i), BF/4(im1)
  Shift2/1 -> delay/1(r), BF/3(re1)
  en/1 -> Counter1/1
  Constant/1 -> Relational/2
  Relational/1 -> Register2/2
  Constant1/1 -> Register2/1
  delay/1(rr) -> BF/1(re2), Twiddle/1(r)
  delay/2(ii) -> BF/2(im2), Twiddle/2(i)
  BF/3(Out1_r) -> delay/4(r1)
  BF/4(Out1_i) -> delay/5(i1)
  Register2/1 -> Delay1/1
  Counter1/1 -> Relational/1, Delay4/1, Twiddle/3(cnt), delay/3(cnt)
  re/1 -> Shift2/1
  im/1 -> Shift3/1
  Twiddle/1(rr) -> Multiplexer/1(r1)
  Twiddle/2(ii) -> Multiplexer/2(i1)
  BF/1(Out2_r) -> Multiplexer/3(r2)
  BF/2(Out2_i) -> Multiplexer/4(i2)
  Delay4/1 -> Multiplexer/5(cnt)
  Multiplexer/1(rr) -> out_re/1
  Multiplexer/2(ii) -> out_im/1
  Delay1/1 -> valid/1

== system sys1/SAR/stream/stream_fft/stage6 ==
  en : Inport
  re : Inport  Port=2
  im : Inport  Port=3
  BF : Subsystem
      settings: PortSchema="{\"entries\":[{\"content\":{\"sides\":[{\"content\":{\"connectorIds\":[\"In1\",\"In2\",\"Out3\",\"Out4\"]},\"type\":\"ConnectorPlacement.EquallySpacedRectSide\",\"uuid\":\"dc9f2664-179f-4a56-867a-12fe61ba91e8\"},{\"content\":{\"connectorIds\":[\"Out1\",\"Out2\",\"In3\",\"In4\"],\"side\":\"RIGHT\"},\"type\":\"ConnectorPlacement.EquallySpacedRectSide\",\"uuid\":\"0b440064-4d1a-4bb1-bd44-91090294f336\"},{\"content\":{\"side\":\"TOP\"},\"type\":\"ConnectorPlacement.EquallySpacedRectSide\",\"uuid\":\"bf93b41b-a3ae-4711-be50-aae2b8452a00\"}]},\"type\":\"ConnectorPlacement.EquallySpacedConnector\",\"uuid\":\"12001bad-0a53-45ef-b6ab-2c1b34cc57fa\"}],\"packageUris\":[\"http://schema.mathworks.com/mf0/Connector/R2020b\"],\"version\":\"1.0\"}"
  Constant : hdlBasic/Constant  const=2^15  gui_display_data_type=Fixed-point  arith_type=Unsigned  n_bits=20  bin_pt=0  preci_type=Single  exp_width=8  frac_width=24  explicit_period=off  period=1  XmcBlockStatus=1  maskContainerNames=tabcontainer1  block_type=constant  block_config=sysgen:Constant_config
  Constant1 : hdlBasic/Constant  const=1  gui_display_data_type=Boolean  arith_type=Boolean  n_bits=16  bin_pt=14  preci_type=Single  exp_width=8  frac_width=24  explicit_period=on  period=ts  XmcBlockStatus=1  maskContainerNames=tabcontainer1  block_type=constant  block_config=sysgen:Constant_config
  Counter1 : hdlBasic/Counter  cnt_type=Free running  cnt_to=Inf  operation=Up  start_count=0  cnt_by_val=1  arith_type=Unsigned  n_bits=20  bin_pt=0  load_pin=off  rst=off  en=on  explicit_period=Explicit  period=ts  use_behavioral_HDL=off  implementation=Fabric  XmcBlockStatus=1  maskContainerNames=group1  block_type=counter  block_config=sysgen:Counter_config  block_width=531  block_height=1023
  Delay1 : hdlBasic/Delay  rst=off  en=off  latency=6  reg_retiming=off  XmcBlockStatus=1  maskContainerNames=group1  block_type=delay  block_config=sysgen:Delay_config
  Delay4 : hdlBasic/Delay  rst=off  en=off  latency=7  reg_retiming=off  XmcBlockStatus=1  maskContainerNames=group1  block_type=delay  block_config=sysgen:Delay_config
  Multiplexer : Subsystem
      settings: PortSchema="{\"entries\":[{\"content\":{\"sides\":[{\"content\":{\"connectorIds\":[\"In1\",\"In2\",\"In3\",\"In4\"]},\"type\":\"ConnectorPlacement.EquallySpacedRectSide\",\"uuid\":\"d39b2674-e61f-4632-a918-ea673b128ff5\"},{\"content\":{\"connectorIds\":[\"Out1\",\"Out2\"],\"side\":\"RIGHT\"},\"type\":\"ConnectorPlacement.EquallySpacedRectSide\",\"uuid\":\"03c9bc0a-e0d2-45eb-9b7a-9d06bc1b3e13\"},{\"content\":{\"connectorIds\":[\"In5\"],\"side\":\"TOP\"},\"type\":\"ConnectorPlacement.EquallySpacedRectSide\",\"uuid\":\"49e788e0-ebb0-431e-96ea-edf312796710\"}]},\"type\":\"ConnectorPlacement.EquallySpacedConnector\",\"uuid\":\"eef61444-07bb-4ce5-a4f8-b8563d493c59\"}],\"packageUris\":[\"http://schema.mathworks.com/mf0/Connector/R2020b\"],\"version\":\"1.0\"}"
  Register2 : hdlBasic/Register  init=0  rst=off  en=on  XmcBlockStatus=1  maskContainerNames=tabcontainer1  block_type=register  block_config=sysgen:Register_config
  Relational : hdlBasic/Relational  mode=a=b  op_type=Bool  en=off  latency=0  XmcBlockStatus=1  maskContainerNames=tabcontainer1  block_type=relational  block_config=sysgen:Relational_config
  Shift2 : hdlBasic/Shift  shift_dir=Right  shift_bits=1  en=off  latency=0  precision=User Defined  arith_type="Signed  (2's comp)"  n_bits=16  bin_pt=0  quantization="Round  (unbiased: +/- Inf)"  overflow=Flag as error  XmcBlockStatus=1  maskContainerNames=group2  block_type=shift  block_config=sysgen:Shift_config
  Shift3 : hdlBasic/Shift  shift_dir=Right  shift_bits=1  en=off  latency=0  precision=User Defined  arith_type="Signed  (2's comp)"  n_bits=16  bin_pt=0  quantization="Round  (unbiased: +/- Inf)"  overflow=Flag as error  XmcBlockStatus=1  maskContainerNames=group2  block_type=shift  block_config=sysgen:Shift_config
  Twiddle : Subsystem
      settings: PortSchema="{\"entries\":[{\"content\":{\"sides\":[{\"content\":{\"connectorIds\":[\"In1\",\"In2\"]},\"type\":\"ConnectorPlacement.EquallySpacedRectSide\",\"uuid\":\"ecfcc33a-c00e-4245-880a-d3e35376b375\"},{\"content\":{\"connectorIds\":[\"Out1\",\"Out2\"],\"side\":\"RIGHT\"},\"type\":\"ConnectorPlacement.EquallySpacedRectSide\",\"uuid\":\"26b6cb3a-d864-4641-9d64-3816f5e3e677\"},{\"content\":{\"connectorIds\":[\"In3\"],\"side\":\"TOP\"},\"type\":\"ConnectorPlacement.EquallySpacedRectSide\",\"uuid\":\"0115c513-98ce-476e-a096-a4849d96f6f0\"}]},\"type\":\"ConnectorPlacement.EquallySpacedConnector\",\"uuid\":\"ace197b1-74a9-4d2b-80b6-f8336c43cac2\"}],\"packageUris\":[\"http://schema.mathworks.com/mf0/Connector/R2020b\"],\"version\":\"1.0\"}"
  delay : Subsystem
      settings: PortSchema="{\"entries\":[{\"content\":{\"sides\":[{\"content\":{\"connectorIds\":[\"In1\",\"In2\"]},\"type\":\"ConnectorPlacement.EquallySpacedRectSide\",\"uuid\":\"ba2590db-591f-426e-a159-0b5b6e6f2a83\"},{\"content\":{\"connectorIds\":[\"Out1\",\"Out2\",\"In4\",\"In5\"],\"side\":\"RIGHT\"},\"type\":\"ConnectorPlacement.EquallySpacedRectSide\",\"uuid\":\"3a7188c9-1b60-4adb-8ab5-3e5ce503b358\"},{\"content\":{\"connectorIds\":[\"In3\"],\"side\":\"TOP\"},\"type\":\"ConnectorPlacement.EquallySpacedRectSide\",\"uuid\":\"d7972a41-1a3e-4417-8334-615e53660bc0\"}]},\"type\":\"ConnectorPlacement.EquallySpacedConnector\",\"uuid\":\"9fe28d71-4153-49dc-89fd-80824351344f\"}],\"packageUris\":[\"http://schema.mathworks.com/mf0/Connector/R2020b\"],\"version\":\"1.0\"}"
  valid : Outport
  out_re : Outport  Port=2
  out_im : Outport  Port=3
  wires:
  Shift3/1 -> BF/4(im1), delay/2(i)
  Shift2/1 -> BF/3(re1), delay/1(r)
  Delay1/1 -> valid/1
  Multiplexer/2(ii) -> out_im/1
  Multiplexer/1(rr) -> out_re/1
  Delay4/1 -> Multiplexer/5(cnt)
  BF/2(Out2_i) -> Multiplexer/4(i2)
  BF/1(Out2_r) -> Multiplexer/3(r2)
  Twiddle/2(ii) -> Multiplexer/2(i1)
  Twiddle/1(rr) -> Multiplexer/1(r1)
  im/1 -> Shift3/1
  re/1 -> Shift2/1
  Counter1/1 -> delay/3(cnt), Twiddle/3(cnt), Delay4/1, Relational/1
  Register2/1 -> Delay1/1
  BF/4(Out1_i) -> delay/5(i1)
  BF/3(Out1_r) -> delay/4(r1)
  delay/2(ii) -> Twiddle/2(i), BF/2(im2)
  delay/1(rr) -> Twiddle/1(r), BF/1(re2)
  Constant1/1 -> Register2/1
  Relational/1 -> Register2/2
  Constant/1 -> Relational/2
  en/1 -> Counter1/1

== system sys1/SAR/stream/stream_fft/stage7 ==
  en : Inport
  re : Inport  Port=2
  im : Inport  Port=3
  BF : Subsystem
      settings: PortSchema="{\"entries\":[{\"content\":{\"sides\":[{\"content\":{\"connectorIds\":[\"In1\",\"In2\",\"Out3\",\"Out4\"]},\"type\":\"ConnectorPlacement.EquallySpacedRectSide\",\"uuid\":\"dc9f2664-179f-4a56-867a-12fe61ba91e8\"},{\"content\":{\"connectorIds\":[\"Out1\",\"Out2\",\"In3\",\"In4\"],\"side\":\"RIGHT\"},\"type\":\"ConnectorPlacement.EquallySpacedRectSide\",\"uuid\":\"0b440064-4d1a-4bb1-bd44-91090294f336\"},{\"content\":{\"side\":\"TOP\"},\"type\":\"ConnectorPlacement.EquallySpacedRectSide\",\"uuid\":\"bf93b41b-a3ae-4711-be50-aae2b8452a00\"}]},\"type\":\"ConnectorPlacement.EquallySpacedConnector\",\"uuid\":\"12001bad-0a53-45ef-b6ab-2c1b34cc57fa\"}],\"packageUris\":[\"http://schema.mathworks.com/mf0/Connector/R2020b\"],\"version\":\"1.0\"}"
  Constant : hdlBasic/Constant  const=2^16  gui_display_data_type=Fixed-point  arith_type=Unsigned  n_bits=20  bin_pt=0  preci_type=Single  exp_width=8  frac_width=24  explicit_period=off  period=1  XmcBlockStatus=1  maskContainerNames=tabcontainer1  block_type=constant  block_config=sysgen:Constant_config
  Constant1 : hdlBasic/Constant  const=1  gui_display_data_type=Boolean  arith_type=Boolean  n_bits=16  bin_pt=14  preci_type=Single  exp_width=8  frac_width=24  explicit_period=on  period=ts  XmcBlockStatus=1  maskContainerNames=tabcontainer1  block_type=constant  block_config=sysgen:Constant_config
  Counter1 : hdlBasic/Counter  cnt_type=Free running  cnt_to=Inf  operation=Up  start_count=0  cnt_by_val=1  arith_type=Unsigned  n_bits=20  bin_pt=0  load_pin=off  rst=off  en=on  explicit_period=Explicit  period=ts  use_behavioral_HDL=off  implementation=Fabric  XmcBlockStatus=1  maskContainerNames=group1  block_type=counter  block_config=sysgen:Counter_config  block_width=531  block_height=1023
  Delay1 : hdlBasic/Delay  rst=off  en=off  latency=6  reg_retiming=off  XmcBlockStatus=1  maskContainerNames=group1  block_type=delay  block_config=sysgen:Delay_config
  Delay4 : hdlBasic/Delay  rst=off  en=off  latency=7  reg_retiming=off  XmcBlockStatus=1  maskContainerNames=group1  block_type=delay  block_config=sysgen:Delay_config
  Multiplexer : Subsystem
      settings: PortSchema="{\"entries\":[{\"content\":{\"sides\":[{\"content\":{\"connectorIds\":[\"In1\",\"In2\",\"In3\",\"In4\"]},\"type\":\"ConnectorPlacement.EquallySpacedRectSide\",\"uuid\":\"d39b2674-e61f-4632-a918-ea673b128ff5\"},{\"content\":{\"connectorIds\":[\"Out1\",\"Out2\"],\"side\":\"RIGHT\"},\"type\":\"ConnectorPlacement.EquallySpacedRectSide\",\"uuid\":\"03c9bc0a-e0d2-45eb-9b7a-9d06bc1b3e13\"},{\"content\":{\"connectorIds\":[\"In5\"],\"side\":\"TOP\"},\"type\":\"ConnectorPlacement.EquallySpacedRectSide\",\"uuid\":\"49e788e0-ebb0-431e-96ea-edf312796710\"}]},\"type\":\"ConnectorPlacement.EquallySpacedConnector\",\"uuid\":\"eef61444-07bb-4ce5-a4f8-b8563d493c59\"}],\"packageUris\":[\"http://schema.mathworks.com/mf0/Connector/R2020b\"],\"version\":\"1.0\"}"
  Register2 : hdlBasic/Register  init=0  rst=off  en=on  XmcBlockStatus=1  maskContainerNames=tabcontainer1  block_type=register  block_config=sysgen:Register_config
  Relational : hdlBasic/Relational  mode=a=b  op_type=Bool  en=off  latency=0  XmcBlockStatus=1  maskContainerNames=tabcontainer1  block_type=relational  block_config=sysgen:Relational_config
  Shift2 : hdlBasic/Shift  shift_dir=Right  shift_bits=1  en=off  latency=0  precision=User Defined  arith_type="Signed  (2's comp)"  n_bits=16  bin_pt=0  quantization="Round  (unbiased: +/- Inf)"  overflow=Flag as error  XmcBlockStatus=1  maskContainerNames=group2  block_type=shift  block_config=sysgen:Shift_config
  Shift3 : hdlBasic/Shift  shift_dir=Right  shift_bits=1  en=off  latency=0  precision=User Defined  arith_type="Signed  (2's comp)"  n_bits=16  bin_pt=0  quantization="Round  (unbiased: +/- Inf)"  overflow=Flag as error  XmcBlockStatus=1  maskContainerNames=group2  block_type=shift  block_config=sysgen:Shift_config
  Twiddle : Subsystem
      settings: PortSchema="{\"entries\":[{\"content\":{\"sides\":[{\"content\":{\"connectorIds\":[\"In1\",\"In2\"]},\"type\":\"ConnectorPlacement.EquallySpacedRectSide\",\"uuid\":\"ecfcc33a-c00e-4245-880a-d3e35376b375\"},{\"content\":{\"connectorIds\":[\"Out1\",\"Out2\"],\"side\":\"RIGHT\"},\"type\":\"ConnectorPlacement.EquallySpacedRectSide\",\"uuid\":\"26b6cb3a-d864-4641-9d64-3816f5e3e677\"},{\"content\":{\"connectorIds\":[\"In3\"],\"side\":\"TOP\"},\"type\":\"ConnectorPlacement.EquallySpacedRectSide\",\"uuid\":\"0115c513-98ce-476e-a096-a4849d96f6f0\"}]},\"type\":\"ConnectorPlacement.EquallySpacedConnector\",\"uuid\":\"ace197b1-74a9-4d2b-80b6-f8336c43cac2\"}],\"packageUris\":[\"http://schema.mathworks.com/mf0/Connector/R2020b\"],\"version\":\"1.0\"}"
  delay : Subsystem
      settings: PortSchema="{\"entries\":[{\"content\":{\"sides\":[{\"content\":{\"connectorIds\":[\"In1\",\"In2\"]},\"type\":\"ConnectorPlacement.EquallySpacedRectSide\",\"uuid\":\"ba2590db-591f-426e-a159-0b5b6e6f2a83\"},{\"content\":{\"connectorIds\":[\"Out1\",\"Out2\",\"In4\",\"In5\"],\"side\":\"RIGHT\"},\"type\":\"ConnectorPlacement.EquallySpacedRectSide\",\"uuid\":\"3a7188c9-1b60-4adb-8ab5-3e5ce503b358\"},{\"content\":{\"connectorIds\":[\"In3\"],\"side\":\"TOP\"},\"type\":\"ConnectorPlacement.EquallySpacedRectSide\",\"uuid\":\"d7972a41-1a3e-4417-8334-615e53660bc0\"}]},\"type\":\"ConnectorPlacement.EquallySpacedConnector\",\"uuid\":\"9fe28d71-4153-49dc-89fd-80824351344f\"}],\"packageUris\":[\"http://schema.mathworks.com/mf0/Connector/R2020b\"],\"version\":\"1.0\"}"
  valid : Outport
  out_re : Outport  Port=2
  out_im : Outport  Port=3
  wires:
  Shift3/1 -> delay/2(i), BF/4(im1)
  Shift2/1 -> delay/1(r), BF/3(re1)
  en/1 -> Counter1/1
  Constant/1 -> Relational/2
  Relational/1 -> Register2/2
  Constant1/1 -> Register2/1
  delay/1(rr) -> BF/1(re2), Twiddle/1(r)
  delay/2(ii) -> BF/2(im2), Twiddle/2(i)
  BF/3(Out1_r) -> delay/4(r1)
  BF/4(Out1_i) -> delay/5(i1)
  Register2/1 -> Delay1/1
  Counter1/1 -> Relational/1, Delay4/1, Twiddle/3(cnt), delay/3(cnt)
  re/1 -> Shift2/1
  im/1 -> Shift3/1
  Twiddle/1(rr) -> Multiplexer/1(r1)
  Twiddle/2(ii) -> Multiplexer/2(i1)
  BF/1(Out2_r) -> Multiplexer/3(r2)
  BF/2(Out2_i) -> Multiplexer/4(i2)
  Delay4/1 -> Multiplexer/5(cnt)
  Multiplexer/1(rr) -> out_re/1
  Multiplexer/2(ii) -> out_im/1
  Delay1/1 -> valid/1
